simulink model "ADCS_origin"  (R2023a)
settings: Solver=VariableStepAuto  StartTime=0.0  StopTime=10.0  RelTol=1e-3
undefined symbols (not defined in the file or in its folder): DiscIntNeverNeededParam
settings Model: DataDictionary=SatelliteTelescope.sldd  Creator=admin  LastModifiedBy=admin

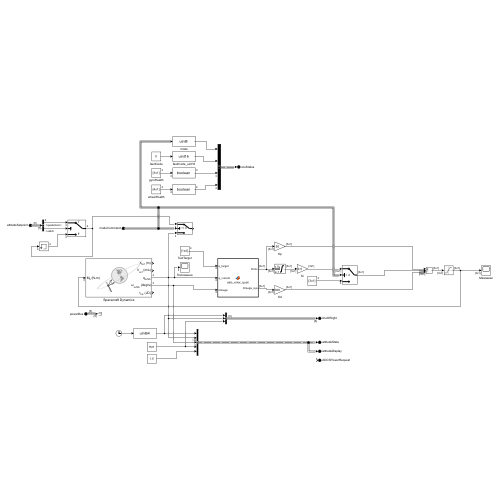
[thumbnail: Simulink's stored preview of the top-level diagram]
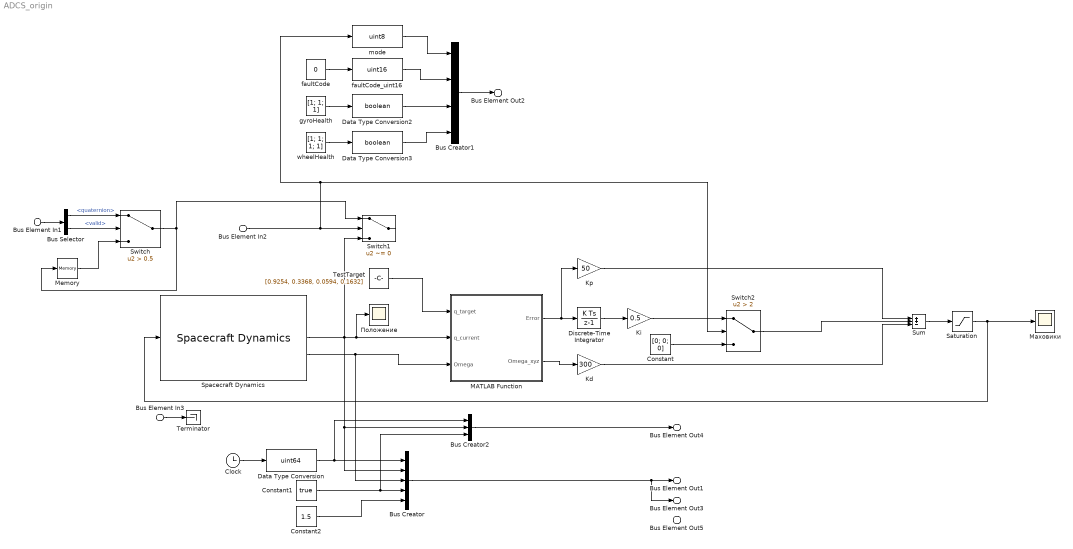
== system ADCS_origin ==
  Bus Element In3 : Inport  PortName=powerBus
  Bus Element In1 : Inport  Port=2  PortName=attitudeSetpoint
  Bus Element In2 : Inport  Port=3  PortName=modeCommand
  Bus Creator : BusCreator  Inputs=5  OutDataTypeStr=Bus: AttitudeState_IF  NonVirtualBus=on
      settings: InheritFromInputs=off
  Bus Creator1 : BusCreator  Inputs=4  OutDataTypeStr=Bus: OcsStatus_IF  NonVirtualBus=on
      settings: InheritFromInputs=off
  Bus Creator2 : BusCreator  Inputs=3  OutDataTypeStr=Bus: LineOfSight_IF
      settings: InheritFromInputs=off
  Bus Selector : BusSelector  OutputSignals=quaternion,valid
  Clock : Clock
  Constant : Constant  Value=[0; 0; 0]
  Constant1 : Constant  Value=true
  Constant2 : Constant  Value=1.5
  Data Type Conversion : DataTypeConversion  OutDataTypeStr=uint64  SaturateOnIntegerOverflow=off  RndMeth=Floor
  Data Type Conversion2 : DataTypeConversion  OutDataTypeStr=boolean  SaturateOnIntegerOverflow=off  RndMeth=Floor
  Data Type Conversion3 : DataTypeConversion  OutDataTypeStr=boolean  SaturateOnIntegerOverflow=off  RndMeth=Floor
  Discrete-Time Integrator : DiscreteIntegrator  SampleTime=0.01  LimitOutput=on  UpperSaturationLimit=0.05  LowerSaturationLimit=-0.05  ICPrevOutput=DiscIntNeverNeededParam  ICPrevScaledInput=DiscIntNeverNeededParam
  Kd : Gain  Gain=300
  Ki : Gain  Gain=0.5
  Kp : Gain  Gain=50
  MATLAB Function : MATLAB Function  TreatAsAtomicUnit=on
  Memory : Memory  InitialCondition=[1, 0, 0, 0]
  Saturation : Saturate  UpperLimit=2  LowerLimit=-2
  Spacecraft Dynamics : SpacecraftDynamics  forcesIn=off  mass=1480  inertia=[1300, 0, 0; 0, 1400, 0; 0, 0, 900]
  Sum : Sum  Inputs=++-
  Switch : Switch  Criteria=u2 > Threshold  Threshold=0.5  SaturateOnIntegerOverflow=off  InputSameDT=off
  Switch1 : Switch  Criteria=u2 ~= 0  SaturateOnIntegerOverflow=off  InputSameDT=off
  Switch2 : Switch  Criteria=u2 > Threshold  Threshold=2  SaturateOnIntegerOverflow=off  InputSameDT=off
  Terminator : Terminator
  TestTarget : Constant  Value=[0.9254, 0.3368, 0.0594, 0.1632]
  faultCode : Constant  Value=0
  faultCode_uint16 : DataTypeConversion  OutDataTypeStr=uint16  SaturateOnIntegerOverflow=off  RndMeth=Floor
  gyroHealth : Constant  Value=[1; 1; 1]
  mode : DataTypeConversion  OutDataTypeStr=uint8  SaturateOnIntegerOverflow=off  RndMeth=Floor
  wheelHealth : Constant  Value=[1; 1; 1; 1]
  Маховики : Scope
  Положение : Scope
  Bus Element Out4 : Outport  PortName=lineOfSight
  Bus Element Out1 : Outport  Port=2  PortName=attitudeState
  Bus Element Out2 : Outport  Port=3  PortName=ocsStatus
  Bus Element Out3 : Outport  Port=4  PortName=attitudeDisplay
  Bus Element Out5 : Outport  Port=5  PortName=ADCSPowerRequest
  wires:
  Spacecraft Dynamics/4 -> Bus Creator/3, MATLAB Function/3(Omega)
  Spacecraft Dynamics/3 -> Bus Creator2/2, Bus Creator/2, Положение/1, MATLAB Function/2(q_current), Switch1/3
  MATLAB Function/1(Error) -> Discrete-Time Integrator/1, Kp/1
  MATLAB Function/2(Omega_xyz) -> Kd/1
  Kp/1 -> Sum/1
  Kd/1 -> Sum/3
  Sum/1 -> Saturation/1
  Saturation/1 -> Маховики/1, Spacecraft Dynamics/1
  Bus Element In1/1 -> Bus Selector/1
  Bus Selector/2 -> Switch/2  "<valid>"
  Bus Selector/1 -> Switch/1  "<quaternion>"
  Memory/1 -> Switch/3
  Switch/1 -> Switch1/1, Memory/1
  Discrete-Time Integrator/1 -> Ki/1
  Ki/1 -> Switch2/1
  Constant/1 -> Switch2/3
  Bus Element In2/1 -> mode/1, Switch2/2, Switch1/2
  Switch2/1 -> Sum/2
  Data Type Conversion/1 -> Bus Creator2/1, Bus Creator/1
  Clock/1 -> Data Type Conversion/1
  Constant1/1 -> Bus Creator2/3, Bus Creator/4
  Constant2/1 -> Bus Creator/5
  Bus Creator/1 -> Bus Element Out3/1, Bus Element Out1/1
  gyroHealth/1 -> Data Type Conversion2/1
  wheelHealth/1 -> Data Type Conversion3/1
  mode/1 -> Bus Creator1/1
  faultCode/1 -> faultCode_uint16/1
  Data Type Conversion2/1 -> Bus Creator1/3
  Data Type Conversion3/1 -> Bus Creator1/4
  Bus Creator1/1 -> Bus Element Out2/1
  Bus Element In3/1 -> Terminator/1
  TestTarget/1 -> MATLAB Function/1(q_target)
  faultCode_uint16/1 -> Bus Creator1/2
  Bus Creator2/1 -> Bus Element Out4/1

== matlab function ADCS_origin/MATLAB Function ==
  data: q_target input; Error output; q_current input; Omega input; Omega_xyz output
function [Error, Omega_xyz] = calc_error_quat(q_target, q_current, Omega)
    q_t = q_target(:)';
    q_c = q_current(:)';
    
    q_err = quatmultiply(quatconj(q_c), q_t);
    
    if q_err(1) < 0
        q_err = -q_err;
    end
    
    Error = rad2deg(2 * q_err(2:4)'); 
    Error = max(min(Error, 5), -5);
    
    Omega_xyz = Omega;
end
